simulink model "EV"  (R2020a)
settings: Solver=VariableStepAuto  StartTime=0.0  StopTime=0.12  RelTol=1e-3
libraries: powerlib x15, powerlib_meascontrol x5, simulink x2
settings Model: Creator=Asus  LastModifiedBy=SHIVAM MAURYA
settings DataIOCC: ReturnWorkspaceOutputs=off

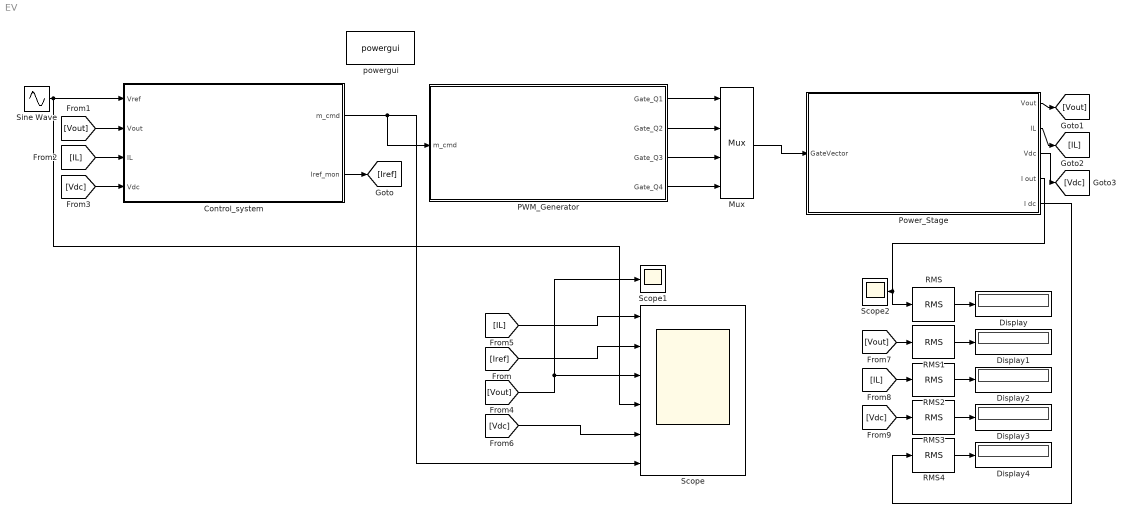
== system EV ==
  Control_system : Subsystem
  Display{,1..4} (5 alike) : Display
  Mux : Mux
  PWM_Generator : Subsystem
  Power_Stage : Subsystem
  RMS{,1..4} (5 alike) : powerlib_meascontrol/Measurements/RMS  TrueRMS=on  Freq=50  RMSInit=0  Ts=1e-6
  Scope : Scope  NumInputPorts=6
  Scope1 : Scope
  Scope2 : Scope
  Sine Wave : Sin  Amplitude=311.127  Frequency=314.159  SampleTime=0
  powergui : powerlib/powergui  Priority=1  SimulationMode=Discrete  SampleTime=1e-6  frequency=60  Iterations=50  frequencyindice=0  Pbase=100e6  ErrMax=1e-4  UnitsV=kV  UnitsW=MW  buscounter=0  FunctionMessages=off  echomessages=off  EnableUseOfTLC=off  CurrentSourceSwitches=off  DisableSnubberDevices=off  DisableRonSwitches=off  DisableVfSwitches=off  DisplayEquations=off  AutomaticDiscreteSolvers=off  SolverType=Tustin/Backward Euler (TBE)  Interpol=off  ExternalGateDelay=off  methode=off  Ts=100  x0status=blocks  SPID=on  SwTol=0  HookPort=off  NonlinearTolerance=1e-4  nMaxIteration=100  ContinueOnMaxIteration=off  RestoreLinks=warning  ResistiveCurrentMeasurement=off  Frange=[0:2:500]  Ylog=off  Xlog=on  ShowGrid=off  save=off  variable=ZData  structure=ScopeVout  ZoomFFT=off  StartTime=0.02  cycles=1  DisplayStyle=1  fundamental=50  FreqAxis=off  MaxFrequency=1000  frequencyindicesteady=1  RmsSteady=1  display=off
  wires:
  PWM_Generator/1(Gate_Q1) -> Mux/1
  PWM_Generator/2(Gate_Q2) -> Mux/2
  PWM_Generator/3(Gate_Q3) -> Mux/3
  PWM_Generator/4(Gate_Q4) -> Mux/4
  Mux/1 -> Power_Stage/1(GateVector)
  Sine Wave/1 -> Scope/4, Control_system/1(Vref)
  Control_system/1(m_cmd) -> Scope/6, PWM_Generator/1(m_cmd)
  Control_system/2(Iref_mon) -> [Iref]
  Power_Stage/1(Vout) -> [Vout]
  Power_Stage/2(IL) -> [IL]
  Power_Stage/3(Vdc) -> [Vdc]
  [Vout] -> Control_system/2(Vout)
  [IL] -> Control_system/3(IL)
  [Vdc] -> Control_system/4(Vdc)
  [IL] -> Scope/1
  [Vout] -> Scope1/1, Scope/3
  [Iref] -> Scope/2
  [Vdc] -> Scope/5
  RMS/1 -> Display/1
  RMS1/1 -> Display1/1
  RMS3/1 -> Display3/1
  RMS2/1 -> Display2/1
  Power_Stage/4(I out) -> RMS/1, Scope2/1
  [Vout] -> RMS1/1
  [IL] -> RMS2/1
  [Vdc] -> RMS3/1
  Power_Stage/5(I dc) -> RMS4/1
  RMS4/1 -> Display4/1

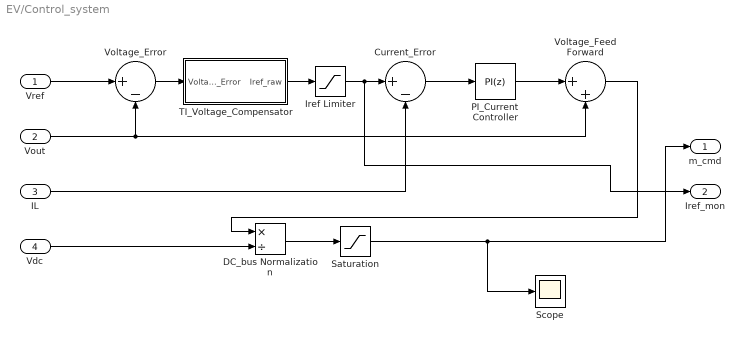
== system EV/Control_system ==
  Vref : Inport
  Vout : Inport  Port=2
  IL : Inport  Port=3
  Vdc : Inport  Port=4
  Current_Error : Sum  Inputs=|+-
  DC_bus Normalization : Product  Inputs=*/
  Iref Limiter : Saturate  UpperLimit=5  LowerLimit=-5
  PI_Current Controller : simulink/Continuous/PID Controller  Controller=PI  Form=Parallel  TimeDomain=Discrete-time  UseExternalTs=off  SampleTime=50e-6  IntegratorMethod=Trapezoidal  FilterMethod=Forward Euler  ControllerParametersSource=internal  P=20  I=6.66e4  D=0  UseFilter=on  N=100  TunerSelectOption=Transfer Function Based (PID Tuner App)  InitialConditionSource=internal  InitialConditionForIntegrator=0  InitialConditionForFilter=0  DifferentiatorICPrevScaledInput=0  ExternalReset=none  TrackingMode=off  Kt=1  LimitOutput=on  UpperSaturationLimit=100  LowerSaturationLimit=-100  LinearizeAsGain=off  AntiWindupMode=clamping  Kb=1  POutMin=[]  POutMax=[]  IOutMin=[]  IOutMax=[]  DOutMin=[]  DOutMax=[]  NOutMin=[]  NOutMax=[]  SumOutMin=[]  SumOutMax=[]  SaturationOutMin=[]  SaturationOutMax=[]  PParamMin=[]  PParamMax=[]  IParamMin=[]  IParamMax=[]  DParamMin=[]  DParamMax=[]  NParamMin=[]  NParamMax=[]  KbParamMin=[]  KbParamMax=[]  KtParamMin=[]  KtParamMax=[]  KbOutMin=[]  KbOutMax=[]  KtOutMin=[]  KtOutMax=[]  IntegratorOutMin=[]  IntegratorOutMax=[]  FilterOutMin=[]  FilterOutMax=[]  SumI1OutMin=[]  SumI1OutMax=[]  SumI2OutMin=[]  SumI2OutMax=[]  SumI3OutMin=[]  SumI3OutMax=[]  SumI4OutMin=[]  SumI4OutMax=[]  SumDOutMin=[]  SumDOutMax=[]  DifferentiatorOutMin=[]  DifferentiatorOutMax=[]  FilterDiffOutCoefMin=[]  FilterDiffOutCoefMax=[]  ReciprocalOutMin=[]  ReciprocalOutMax=[]  SumDenOutMin=[]  SumDenOutMax=[]  SumNumOutMin=[]  SumNumOutMax=[]  DivideOutMin=[]  DivideOutMax=[]  UdiffTsProdOutMin=[]  UdiffTsProdOutMax=[]  NTsProdOutMin=[]  NTsProdOutMax=[]  UintegralTsProdOutMin=[]  UintegralTsProdOutMax=[]  UngainTsProdOutMin=[]  UngainTsProdOutMax=[]  IntegratorContinuousStateAttributes=''  IntegratorStateMustResolveToSignalObject=off  IntegratorRTWStateStorageClass=Auto  FilterContinuousStateAttributes=''  FilterStateMustResolveToSignalObject=off  FilterRTWStateStorageClass=Auto  ParallelPVariant=InternalParameters  IdealPVariant=Disabled  IVariant=InternalParameters  DVariant=Disabled  IntegratorVariant=Discrete  SatVariant=Enabled  AWVariant=DiscClampingParallel  PCopyVariant=Disabled  TRVariant=Disabled  FdbkBlocksVariant=Feedback  IdealPFdbkVariant=Passthrough  SatFdbkVariant=Passthrough  DerivativeFilterVariant=Disabled  NVariant=Disabled  NCopyVariant=Disabled_SignalSpec  FilterICVariant=Disabled  IntegratorICVariant=InternalICs  ExternalResetVariant=Disabled  TRSumVariant=Passthrough  SumFdbkVariant=Enabled  SumVariant=Sum_PI  TsampFilterVariant=InternalTs  TsampNgainVariant=Passthrough  TsampIntegralVariant=Passthrough
  Saturation : Saturate  UpperLimit=0.95  LowerLimit=-0.95
  Scope : Scope
  TI_Voltage_Compensator : Subsystem
  Voltage_Error : Sum  Inputs=|+-
  Voltage_Feed Forward : Sum  Inputs=|++
  m_cmd : Outport
  Iref_mon : Outport  Port=2
  wires:
  Vref/1 -> Voltage_Error/1
  Vout/1 -> Voltage_Feed Forward/2, Voltage_Error/2
  IL/1 -> Current_Error/2
  Current_Error/1 -> PI_Current Controller/1
  PI_Current Controller/1 -> Voltage_Feed Forward/1
  Voltage_Feed Forward/1 -> DC_bus Normalization/1
  Vdc/1 -> DC_bus Normalization/2
  DC_bus Normalization/1 -> Saturation/1
  Saturation/1 -> Scope/1, m_cmd/1
  Iref Limiter/1 -> Iref_mon/1, Current_Error/1
  Voltage_Error/1 -> TI_Voltage_Compensator/1(Voltage_Error)
  TI_Voltage_Compensator/1(Iref_raw) -> Iref Limiter/1

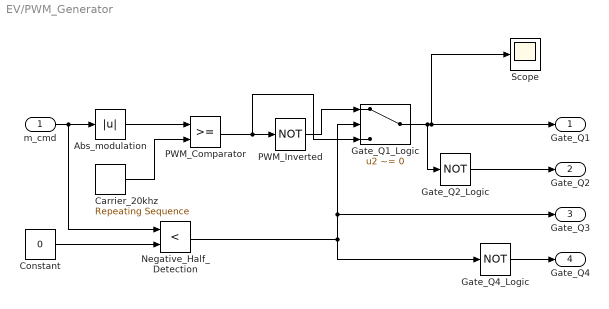
== system EV/PWM_Generator ==
  m_cmd : Inport
  Abs_modulation : Abs
  Carrier_20khz : simulink/Sources/Repeating Sequence  rep_seq_t=[0 25e-6 50e-6]  rep_seq_y=[0 1 0]
  Constant : Constant  Value=0
  Gate_Q1_Logic : Switch  Criteria=u2 ~= 0
  Gate_Q2_Logic : Logic  Operator=NOT  AllPortsSameDT=off  OutDataTypeStr=boolean
  Gate_Q4_Logic : Logic  Operator=NOT  AllPortsSameDT=off  OutDataTypeStr=boolean
  Negative_Half_Detection : RelationalOperator  Operator=<  OutDataTypeStr=boolean  RndMeth=Simplest
  PWM_Comparator : RelationalOperator  OutDataTypeStr=boolean  RndMeth=Simplest
  PWM_Inverted : Logic  Operator=NOT  AllPortsSameDT=off  OutDataTypeStr=boolean
  Scope : Scope
  Gate_Q1 : Outport
  Gate_Q2 : Outport  Port=2
  Gate_Q3 : Outport  Port=3
  Gate_Q4 : Outport  Port=4
  wires:
  Abs_modulation/1 -> PWM_Comparator/1
  Carrier_20khz/1 -> PWM_Comparator/2
  m_cmd/1 -> Negative_Half_Detection/1, Abs_modulation/1
  Constant/1 -> Negative_Half_Detection/2
  PWM_Comparator/1 -> Gate_Q1_Logic/3, PWM_Inverted/1
  PWM_Inverted/1 -> Gate_Q1_Logic/1
  Negative_Half_Detection/1 -> Gate_Q1_Logic/2, Gate_Q3/1, Gate_Q4_Logic/1
  Gate_Q1_Logic/1 -> Gate_Q2_Logic/1, Scope/1, Gate_Q1/1
  Gate_Q2_Logic/1 -> Gate_Q2/1
  Gate_Q4_Logic/1 -> Gate_Q4/1

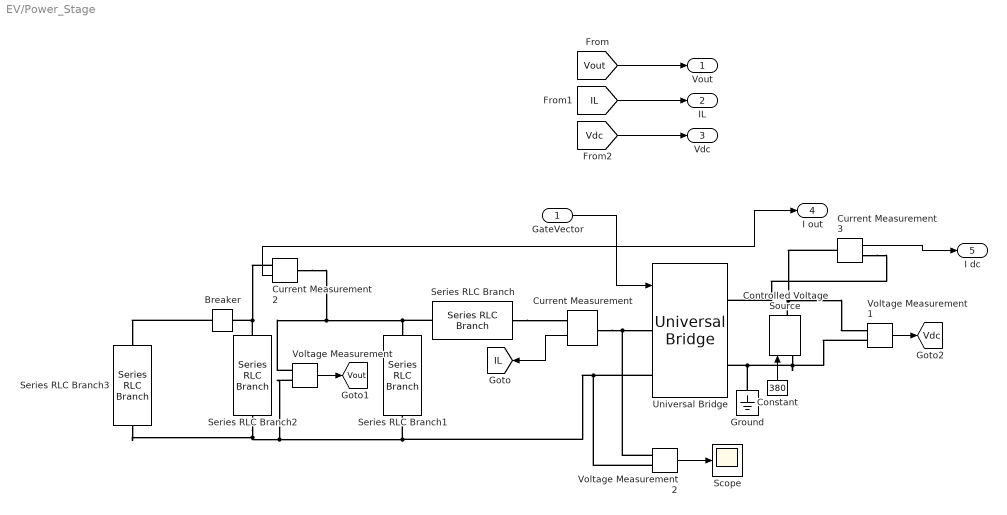
== system EV/Power_Stage ==
  GateVector : Inport
  Breaker : powerlib/Elements/Breaker  InitialState=0  SwitchingTimes=[0.04 0.08]  External=off  BreakerResistance=0.01  SnubberResistance=1e6  SnubberCapacitance=inf  Measurements=None  MoreParameters=on  NoBreakLoop=off
  Constant : Constant  Value=380
  Controlled Voltage Source : powerlib/Electrical Sources/Controlled Voltage Source  Initialize=on  Source_Type=DC  Amplitude=380  Phase=0  Frequency=0  Measurements=None
  Current Measurement : powerlib/Measurements/Current Measurement  PhasorSimulation=off  OutputType=Complex  PSBequivalent=0
  Current Measurement2 : powerlib/Measurements/Current Measurement  PhasorSimulation=off  OutputType=Complex  PSBequivalent=0
  Current Measurement3 : powerlib/Measurements/Current Measurement  PhasorSimulation=off  OutputType=Complex  PSBequivalent=0
  Ground : powerlib/Elements/Ground  LConnTagsString=a
  Scope : Scope
  Series RLC Branch : powerlib/Elements/Series RLC Branch  LConnTagsString=__new0  RConnTagsString=__new0  BranchType=L  Resistance=1  Inductance=3e-3  SetiL0=off  InitialCurrent=0  Capacitance=1e-6  Setx0=off  InitialVoltage=0  Measurements=None
  Series RLC Branch1 : powerlib/Elements/Series RLC Branch  LConnTagsString=__new0  RConnTagsString=__new0  BranchType=C  Resistance=1  Inductance=1e-3  SetiL0=off  InitialCurrent=0  Capacitance=20e-6  Setx0=off  InitialVoltage=0  Measurements=None
  Series RLC Branch2 : powerlib/Elements/Series RLC Branch  LConnTagsString=__new0  RConnTagsString=__new0  BranchType=R  Resistance=100  Inductance=1e-3  SetiL0=off  InitialCurrent=0  Capacitance=1e-6  Setx0=off  InitialVoltage=0  Measurements=None
  Series RLC Branch3 : powerlib/Elements/Series RLC Branch  LConnTagsString=__new0  RConnTagsString=__new0  BranchType=R  Resistance=560  Inductance=1e-3  SetiL0=off  InitialCurrent=0  Capacitance=1e-6  Setx0=off  InitialVoltage=0  Measurements=None
  Universal Bridge : powerlib/Power Electronics/Universal Bridge  Arms=2  SnubberResistance=1e5  SnubberCapacitance=inf  Device=IGBT / Diodes  Ron=1e-3  Lon=0  ForwardVoltages="[  0  0  ]"  ForwardVoltage=0  GTOparameters=[ 10e-6 , 20e-6 ]  IGBTparameters=[ 1e-6 , 2e-6 ]  Measurements=None  Measurements_2=None  converterType=Rectifier
  Voltage Measurement : powerlib/Measurements/Voltage Measurement  PhasorSimulation=off  OutputType=Complex  PSBequivalent=0
  Voltage Measurement1 : powerlib/Measurements/Voltage Measurement  PhasorSimulation=off  OutputType=Complex  PSBequivalent=0
  Voltage Measurement2 : powerlib/Measurements/Voltage Measurement  PhasorSimulation=off  OutputType=Complex  PSBequivalent=0
  Vout : Outport
  IL : Outport  Port=2
  Vdc : Outport  Port=3
  I out : Outport  Port=4
  I dc : Outport  Port=5
  tag scope: IL=global, Vdc=global, Vout=global
  wires:
  GateVector/1 -> Universal Bridge/1
  Current Measurement/1 -> [IL]
  Voltage Measurement/1 -> [Vout]
  Voltage Measurement1/1 -> [Vdc]
  [Vout] -> Vout/1
  [IL] -> IL/1
  [Vdc] -> Vdc/1
  Constant/1 -> Controlled Voltage Source/1
  Current Measurement2/1 -> I out/1
  Current Measurement3/1 -> I dc/1
  Voltage Measurement2/1 -> Scope/1
  connections:
  Controlled Voltage Source/RConn1 -- Current Measurement3/LConn1 -- Voltage Measurement1/LConn1
  Ground/LConn1 -- Universal Bridge/RConn2 -- Controlled Voltage Source/LConn1 -- Voltage Measurement1/LConn2
  Current Measurement/LConn1 -- Voltage Measurement2/LConn1 -- Universal Bridge/LConn1
  Series RLC Branch/RConn1 -- Current Measurement/RConn1
  Series RLC Branch/LConn1 -- Current Measurement2/LConn1 -- Voltage Measurement/LConn1 -- Series RLC Branch1/LConn1
  Universal Bridge/LConn2 -- Voltage Measurement2/LConn2 -- Series RLC Branch3/RConn1 -- Series RLC Branch2/RConn1 -- Voltage Measurement/LConn2 -- Series RLC Branch1/RConn1
  Breaker/LConn1 -- Series RLC Branch3/LConn1
  Series RLC Branch2/LConn1 -- Current Measurement2/RConn1 -- Breaker/RConn1
  Current Measurement3/RConn1 -- Universal Bridge/RConn1

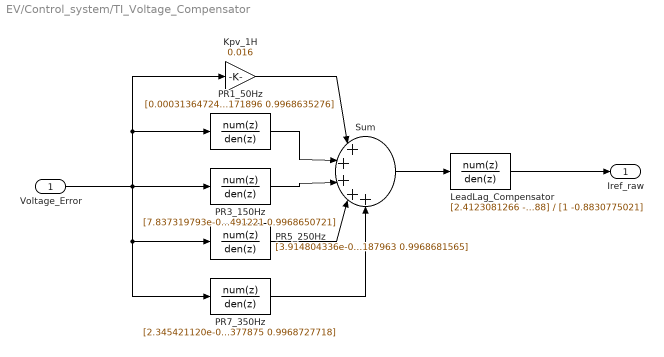
== system EV/Control_system/TI_Voltage_Compensator ==
  Voltage_Error : Inport
  Kpv_1H : Gain  Gain=0.016
  LeadLag_Compensator : DiscreteTransferFcn  Numerator=[2.4123081266 -2.2953856288]  Denominator=[1 -0.8830775021]  SampleTime=50e-6
  PR1_50Hz : DiscreteTransferFcn  Numerator=[0.0003136472421 0 -0.0003136472421]  Denominator=[1 -1.9966171896 0.9968635276]  SampleTime=50e-6
  PR3_150Hz : DiscreteTransferFcn  Numerator=[7.837319793e-05 0 -7.837319793e-05]  Denominator=[1 -1.9946491221 0.9968650721]  SampleTime=50e-6
  PR5_250Hz : DiscreteTransferFcn  Numerator=[3.914804336e-05 0 -3.914804336e-05]  Denominator=[1 -1.9907187963 0.9968681565]  SampleTime=50e-6
  PR7_350Hz : DiscreteTransferFcn  Numerator=[2.345421120e-05 0 -2.345421120e-05]  Denominator=[1 -1.9848377875 0.9968727718]  SampleTime=50e-6
  Sum : Sum  Inputs=|+++++
  Iref_raw : Outport
  wires:
  Voltage_Error/1 -> PR7_350Hz/1, PR5_250Hz/1, Kpv_1H/1, PR1_50Hz/1, PR3_150Hz/1
  Kpv_1H/1 -> Sum/1
  PR1_50Hz/1 -> Sum/2
  PR3_150Hz/1 -> Sum/3
  PR5_250Hz/1 -> Sum/4
  PR7_350Hz/1 -> Sum/5
  Sum/1 -> LeadLag_Compensator/1
  LeadLag_Compensator/1 -> Iref_raw/1
